simulink model "part1_ballbeam"  (R2024b)
settings: Solver=ode45  StartTime=0.0  StopTime=10  MaxStep=0.005  RelTol=1e-8  AbsTol=1e-10
model workspace (MAT data in the model file):
  A_cl = [0  1  0  0; 0  0  1  0; 0  0  0  1; -16  -32  -24  -8]
  B = 0.714285714286
  B_cl = [0  0  0  0  0; 0  0  0  0  0; 0  0  0  0  0; 16  32  24  8  1]
  C_cl = [1 0 0 0]
  D_cl = [0 0 0 0 0]
  J = 0.02
  Jb = 9.9e-06
  Kc = [16 32 24 8]
  R = 0.015
  dr0 = 0
  dtheta0 = 0
  g = 9.81
  m = 0.11
  meas_step = 1
  meas_t0 = 0
  n = 4
  p = 2
  r0 = 0.2
  r_d0 = 0
  r_d1 = 0
  t_ref = 1
  t_stop = 10
  t_stop_plant = 3
  t_u = 0.5
  t_unit = 's'
  theta0 = 0
  ts = 4.54205769121
  u0 = 0.21582
  u_name = 'u [N m]'
  u_step = 0.001
  v_name = 'v [m/s^4]'
  x_names = {'r [m]', 'dr/dt [m/s]', '\theta [rad]', 'd\theta/dt [rad/s]'}
  xs = 9.08411538241
  y_name = 'r [m]'
  z0 = [0.2; 0; 0; 0]
settings Model: Creator=larss  LastModifiedBy=matiasgarcia

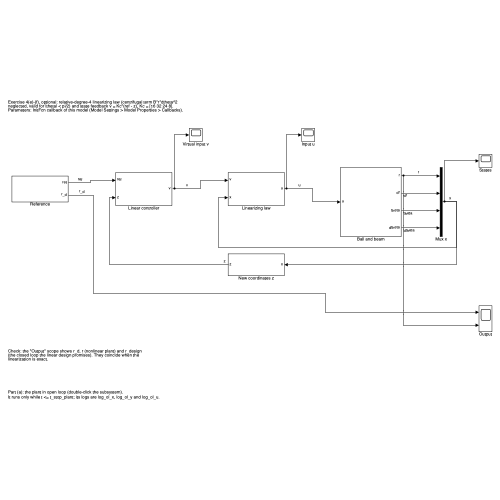
[thumbnail: Simulink's stored preview of the top-level diagram]
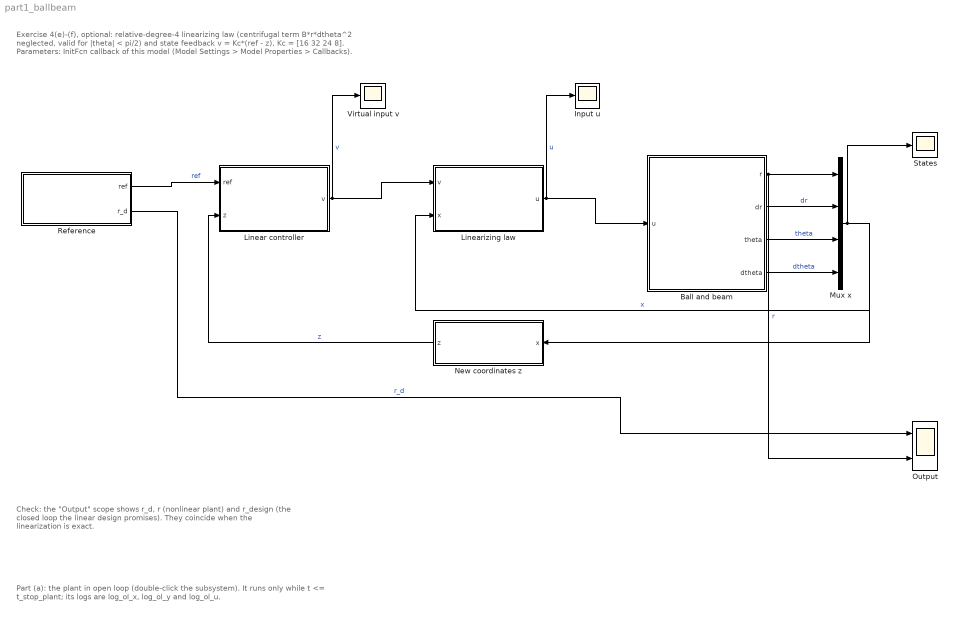
== system part1_ballbeam ==
  note: Exercise 4(e)-(f), optional: relative-degree-4 linearizing law (centrifugal term B*r*dtheta^2
      | neglected, valid for |theta| < pi/2) and state feedback v = Kc*(ref - z), Kc = [16 32 24 8].
      | Parameters: InitFcn callback of this model (Model Settings > Model Properties > Callbacks).
  note: Check: the "Output" scope shows r_d, r (nonlinear plant) and r_design
      | (the closed loop the linear design promises). They coincide when the
      | linearization is exact.
  note: Part (a): the plant in open loop (double-click the subsystem).
      | It runs only while t <= t_stop_plant; its logs are log_ol_x, log_ol_y and log_ol_u.
  Ball and beam : Subsystem
  Input u : Scope
  Linear controller : Subsystem
  Linearizing law : Subsystem
  Mux x : Mux
  New coordinates z : Subsystem
  Output : Scope  NumInputPorts=2
  Reference : Subsystem
  States : Scope
  Virtual input v : Scope
  wires:
  Reference/1(ref) -> Linear controller/1(ref)  "ref"
  Reference/2(r_d) -> Output/1  "r_d"
  Linear controller/1(v) -> Linearizing law/1(v), Virtual input v/1  "v"
  Linearizing law/1(u) -> Ball and beam/1(u), Input u/1  "u"
  Ball and beam/1(r) -> Mux x/1, Output/2  "r"
  Ball and beam/2(dr) -> Mux x/2  "dr"
  Ball and beam/3(theta) -> Mux x/3  "theta"
  Ball and beam/4(dtheta) -> Mux x/4  "dtheta"
  Mux x/1 -> Linearizing law/2(x), New coordinates z/1(x), States/1  "x"
  New coordinates z/1(z) -> Linear controller/2(z)  "z"

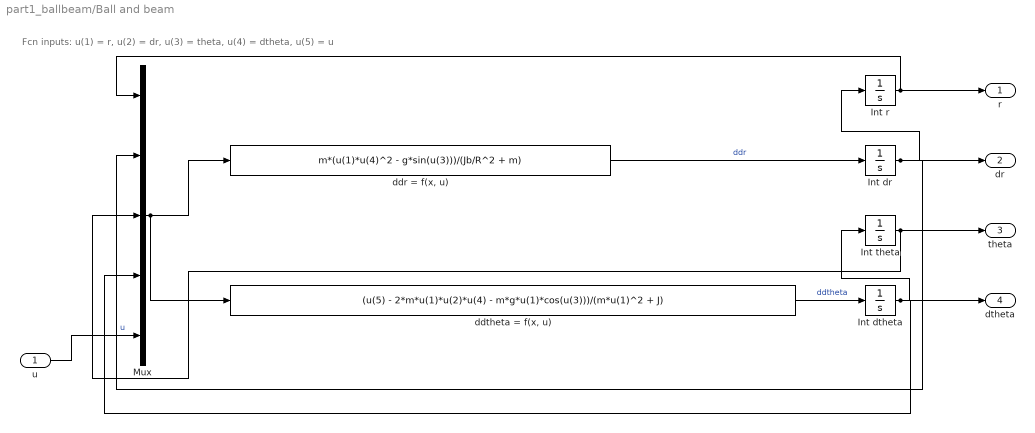
== system part1_ballbeam/Ball and beam ==
  note: Fcn inputs: u(1) = r, u(2) = dr, u(3) = theta, u(4) = dtheta, u(5) = u
  u : Inport
  Int dr : Integrator  InitialCondition=dr0
  Int dtheta : Integrator  InitialCondition=dtheta0
  Int r : Integrator  InitialCondition=r0
  Int theta : Integrator  InitialCondition=theta0
  Mux : Mux  Inputs=5
  "ddr = f(x, u)" : Fcn  Expr=m*(u(1)*u(4)^2 - g*sin(u(3)))/(Jb/R^2 + m)
  "ddtheta = f(x, u)" : Fcn  Expr=(u(5) - 2*m*u(1)*u(2)*u(4) - m*g*u(1)*cos(u(3)))/(m*u(1)^2 + J)
  r : Outport
  dr : Outport  Port=2
  theta : Outport  Port=3
  dtheta : Outport  Port=4
  wires:
  Int r/1 -> r/1, Mux/1
  Int dr/1 -> Int r/1, dr/1, Mux/2
  Mux/1 -> "ddr = f(x, u)"/1, "ddtheta = f(x, u)"/1
  "ddr = f(x, u)"/1 -> Int dr/1  "ddr"
  Int theta/1 -> theta/1, Mux/3
  Int dtheta/1 -> Int theta/1, dtheta/1, Mux/4
  "ddtheta = f(x, u)"/1 -> Int dtheta/1  "ddtheta"
  u/1 -> Mux/5  "u"

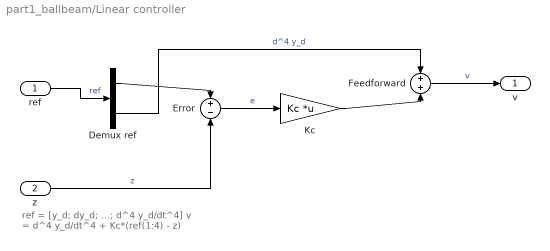
== system part1_ballbeam/Linear controller ==
  note: ref = [y_d; dy_d; ...; d^4 y_d/dt^4]
      | v = d^4 y_d/dt^4 + Kc*(ref(1:4) - z)
  ref : Inport
  z : Inport  Port=2
  Demux ref : Demux  Outputs=[4 1]
  Error : Sum  Inputs=+-
  Feedforward : Sum
  Kc : Gain  Gain=Kc  Multiplication=Matrix(K*u) (u vector)
  v : Outport
  wires:
  ref/1 -> Demux ref/1  "ref"
  Demux ref/1 -> Error/1
  z/1 -> Error/2  "z"
  Error/1 -> Kc/1  "e"
  Kc/1 -> Feedforward/2
  Demux ref/2 -> Feedforward/1  "d^4 y_d"
  Feedforward/1 -> v/1  "v"

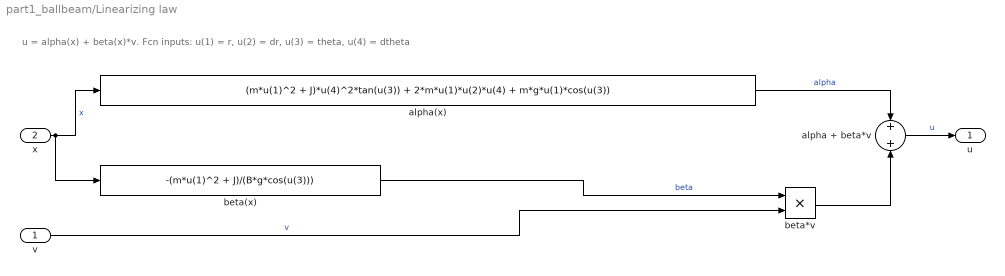
== system part1_ballbeam/Linearizing law ==
  note: u = alpha(x) + beta(x)*v. Fcn inputs: u(1) = r, u(2) = dr, u(3) = theta, u(4) = dtheta
  v : Inport
  x : Inport  Port=2
  alpha + beta*v : Sum
  alpha(x) : Fcn  Expr=(m*u(1)^2 + J)*u(4)^2*tan(u(3)) + 2*m*u(1)*u(2)*u(4) + m*g*u(1)*cos(u(3))
  beta(x) : Fcn  Expr=-(m*u(1)^2 + J)/(B*g*cos(u(3)))
  beta*v : Product
  u : Outport
  wires:
  x/1 -> alpha(x)/1, beta(x)/1  "x"
  beta(x)/1 -> beta*v/1  "beta"
  v/1 -> beta*v/2  "v"
  alpha(x)/1 -> alpha + beta*v/1  "alpha"
  beta*v/1 -> alpha + beta*v/2
  alpha + beta*v/1 -> u/1  "u"

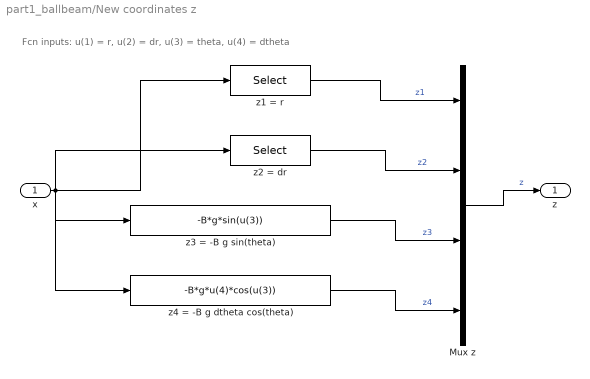
== system part1_ballbeam/New coordinates z ==
  note: Fcn inputs: u(1) = r, u(2) = dr, u(3) = theta, u(4) = dtheta
  x : Inport
  Mux z : Mux
  z1 = r : Selector  InputPortWidth=4  IndexOptions=Index vector (dialog)  Indices=1  OutputSizes=1
  z2 = dr : Selector  InputPortWidth=4  IndexOptions=Index vector (dialog)  Indices=2  OutputSizes=1
  z3 = -B g sin(theta) : Fcn  Expr=-B*g*sin(u(3))
  z4 = -B g dtheta cos(theta) : Fcn  Expr=-B*g*u(4)*cos(u(3))
  z : Outport
  wires:
  x/1 -> z1 = r/1, z2 = dr/1, z3 = -B g sin(theta)/1, z4 = -B g dtheta cos(theta)/1
  z1 = r/1 -> Mux z/1  "z1"
  z2 = dr/1 -> Mux z/2  "z2"
  z3 = -B g sin(theta)/1 -> Mux z/3  "z3"
  z4 = -B g dtheta cos(theta)/1 -> Mux z/4  "z4"
  Mux z/1 -> z/1  "z"

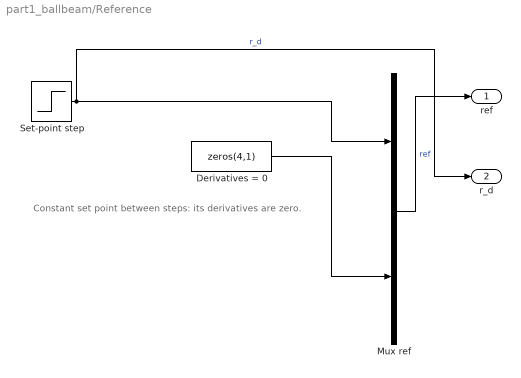
== system part1_ballbeam/Reference ==
  note: Constant set point between steps: its derivatives are zero.
  Derivatives = 0 : Constant  Value=zeros(4,1)
  Mux ref : Mux  Inputs=2
  Set-point step : Step  Time=t_ref  Before=r_d0  After=r_d1  SampleTime=0
  ref : Outport
  r_d : Outport  Port=2
  wires:
  Set-point step/1 -> Mux ref/1, r_d/1  "r_d"
  Derivatives = 0/1 -> Mux ref/2
  Mux ref/1 -> ref/1  "ref"
